simulink model "B1_Acquisition"  (R2022b)
settings: Solver=FixedStepDiscrete  StartTime=0.0  StopTime=30  FixedStep=Ts  RelTol=1e-3
values from neighbouring files (symbols this model uses):
  Ts = 0.01    [build_B2_AutoHeadlamp.m]    (also in build_B3_AHB.m)
undefined symbols (not defined in the file or in its folder): LUX_MAX, T_ABSENT, T_DEB, T_RECOVER, TAU_LUX
settings Model: Creator=LENOVO  LastModifiedBy=LENOVO

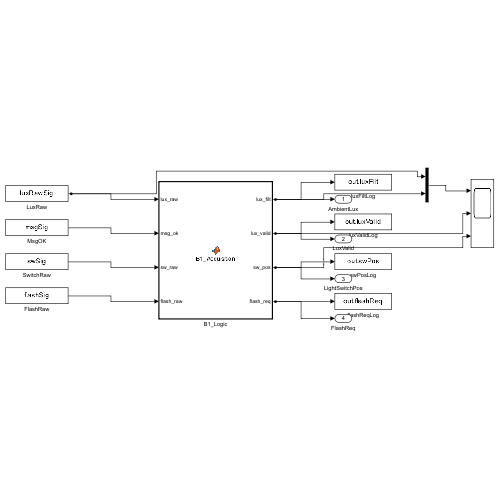
[thumbnail: Simulink's stored preview of the top-level diagram]
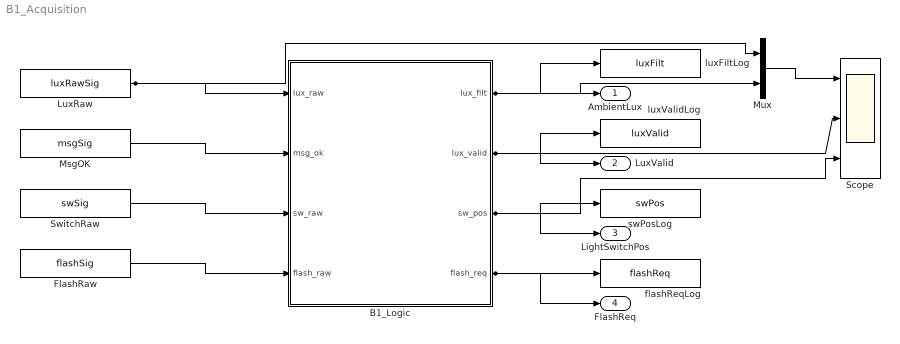
== system B1_Acquisition ==
  B1_Logic : MATLAB Function  TreatAsAtomicUnit=on
  FlashRaw : FromWorkspace  VariableName=flashSig  SampleTime=Ts  Interpolate=off  OutputAfterFinalValue=Holding final value
  LuxRaw : FromWorkspace  VariableName=luxRawSig  SampleTime=Ts  OutputAfterFinalValue=Holding final value
  MsgOK : FromWorkspace  VariableName=msgSig  SampleTime=Ts  Interpolate=off  OutputAfterFinalValue=Holding final value
  Mux : Mux  Inputs=2
  Scope : Scope  NumInputPorts=3
  SwitchRaw : FromWorkspace  VariableName=swSig  SampleTime=Ts  Interpolate=off  OutputAfterFinalValue=Holding final value
  flashReqLog : ToWorkspace  VariableName=flashReq  SaveFormat=Timeseries  SampleTime=-1
  luxFiltLog : ToWorkspace  VariableName=luxFilt  SaveFormat=Timeseries  SampleTime=-1
  luxValidLog : ToWorkspace  VariableName=luxValid  SaveFormat=Timeseries  SampleTime=-1
  swPosLog : ToWorkspace  VariableName=swPos  SaveFormat=Timeseries  SampleTime=-1
  AmbientLux : Outport
  LuxValid : Outport  Port=2
  LightSwitchPos : Outport  Port=3
  FlashReq : Outport  Port=4
  wires:
  LuxRaw/1 -> B1_Logic/1(lux_raw), Mux/1
  MsgOK/1 -> B1_Logic/2(msg_ok)
  SwitchRaw/1 -> B1_Logic/3(sw_raw)
  FlashRaw/1 -> B1_Logic/4(flash_raw)
  B1_Logic/1(lux_filt) -> luxFiltLog/1, AmbientLux/1, Mux/2
  B1_Logic/2(lux_valid) -> luxValidLog/1, LuxValid/1, Scope/2
  B1_Logic/3(sw_pos) -> swPosLog/1, LightSwitchPos/1, Scope/3
  B1_Logic/4(flash_req) -> flashReqLog/1, FlashReq/1
  Mux/1 -> Scope/1

== matlab function B1_Acquisition/B1_Logic ==
  data: lux_raw input; lux_filt output; msg_ok input; sw_raw input; flash_raw input; lux_valid output; sw_pos output; flash_req output; Ts parameter; TAU_LUX parameter; LUX_MAX parameter; T_ABSENT parameter; T_RECOVER parameter; T_DEB parameter
function [lux_filt, lux_valid, sw_pos, flash_req] = B1_Acquisition(lux_raw, msg_ok, sw_raw, flash_raw, Ts, TAU_LUX, LUX_MAX, T_ABSENT, T_RECOVER, T_DEB)
%#codegen
% B1 - Acquisition et filtrage des entrees
%   lux_raw   : mesure brute du capteur de luminosite [lux]
%   msg_ok    : 1 si le message du capteur est recu a ce pas (bus CAN)
%   sw_raw    : position brute du commodo (0 OFF, 1 AUTO, 2 POSITION, 3 CROISEMENT)
%   flash_raw : contact brut du levier d'appel de phares
persistent init yf valid absent_cnt good_cnt sw_last sw_cnt sw_out fl_last fl_cnt fl_out
if isempty(init)
    init = true; yf = lux_raw; valid = true; absent_cnt = 0; good_cnt = 0;
    sw_last = sw_raw; sw_cnt = 0; sw_out = sw_raw;
    fl_last = flash_raw; fl_cnt = 0; fl_out = flash_raw;
end

% ---------- 1) Diagnostic du capteur de luminosite (REQ-LSC-09)
in_range = (lux_raw >= 0) && (lux_raw <= LUX_MAX);
if msg_ok
    absent_cnt = 0;
else
    absent_cnt = min(absent_cnt + Ts, 100);
end
absent = absent_cnt > T_ABSENT + Ts/2;          % message absent depuis plus de 500 ms
if ~in_range || absent
    valid = false; good_cnt = 0;                % defaut detecte immediatement
elseif msg_ok
    good_cnt = min(good_cnt + Ts, 100);
    if good_cnt > T_RECOVER + Ts/2              % retour a la normale apres 1 s de mesures correctes
        valid = true;
    end
end

% ---------- 2) Filtre passe-bas du 1er ordre (NFR-04), fige si mesure non fiable
if in_range && msg_ok
    if lux_raw < 0.2 * yf                       % chute brutale > 80 % (entree de tunnel) :
        yf = lux_raw;                           % suivi immediat, sinon le filtre retarde B2 (REQ-LSC-08)
    else
        a = Ts / (TAU_LUX + Ts);
        yf = yf + a * (lux_raw - yf);
    end
end

% ---------- 3) Anti-rebond du commodo (NFR-04 / REQ-LSC-02)
if sw_raw ~= sw_last
    sw_last = sw_raw; sw_cnt = 0;               % la position bouge : on recommence
else
    sw_cnt = min(sw_cnt + Ts, 100);
    if sw_cnt > T_DEB - Ts/2
        sw_out = sw_raw;                        % stable depuis 50 ms : on valide
    end
end

% ---------- 4) Anti-rebond de l'appel de phares
if flash_raw ~= fl_last
    fl_last = flash_raw; fl_cnt = 0;
else
    fl_cnt = min(fl_cnt + Ts, 100);
    if fl_cnt > T_DEB - Ts/2
        fl_out = flash_raw;
    end
end

lux_filt  = yf;
lux_valid = valid;
sw_pos    = sw_out;
flash_req = fl_out;
